simulink library "Transmission_Lib"  (R2025a)
settings: Solver=ode45  StartTime=0.0  StopTime=10.0  RelTol=1e-3  EnableMultiTasking=on
undefined symbols (not defined in the file): DCT_Param
libraries: fl_lib x45, nesl_utility x25, sdl_lib x18
(part 2 of 2)

== system Transmission_Lib/Detailed/Gears/Actu 6 ==
  p : Inport
  Actuation force (N) : Gain  Gain=10  SaturateOnIntegerOverflow=on  OutDataTypeStr=Inherit: Same as input  ParamDataTypeStr=Inherit: Same as input
  Ideal Force Source : fl_lib/Mechanical/Mechanical Sources/Ideal Force Source
  Mass : fl_lib/Mechanical/Translational Elements/Mass  mass=0.5 kg  num_ports=foundation.enum.numPorts2.one  v_specify=on  v_priority=High  v=0 m/s  v_nominal_specify=off  v_nominal_value=1  v_nominal_unit=m/s  f_specify=off  f_priority=High  f=0 N  f_nominal_specify=off  f_nominal_value=1  f_nominal_unit=N
  Mechanical Translational Reference : fl_lib/Mechanical/Translational Elements/Mechanical Translational Reference
  Rate Transition : RateTransition
  Simulink-PS Converter : nesl_utility/Simulink-PS Converter  PhysicalDomain=network_engine_domain  SubClassName=ps_input  LeftPortType=input  RightPortType=output  PseudoPeriodic=off  Frequencies=[]  NoiseDistribution=none  NoiseParameters=[]  Unit=1  AffineConversion=off  FilteringAndDerivatives=zero  SimscapeFilterOrder=1  InputFilterTimeConstant=0.005  UdotUserProvided=0
  S : PMIOPort  Side=Right
  wires:
  Rate Transition/1 -> Simulink-PS Converter/1
  Actuation force (N)/1 -> Rate Transition/1
  p/1 -> Actuation force (N)/1
  connections:
  Simulink-PS Converter/RConn1 -- Ideal Force Source/RConn1
  Mass/LConn1 -- S/RConn1 -- Ideal Force Source/LConn1
  Ideal Force Source/RConn2 -- Mechanical Translational Reference/LConn1

== system Transmission_Lib/Detailed/Gears/Actu R ==
  p : Inport
  Actuation force (N) : Gain  Gain=10  SaturateOnIntegerOverflow=on  OutDataTypeStr=Inherit: Same as input  ParamDataTypeStr=Inherit: Same as input
  Ideal Force Source : fl_lib/Mechanical/Mechanical Sources/Ideal Force Source
  Mass : fl_lib/Mechanical/Translational Elements/Mass  mass=0.5 kg  num_ports=foundation.enum.numPorts2.one  v_specify=on  v_priority=High  v=0 m/s  v_nominal_specify=off  v_nominal_value=1  v_nominal_unit=m/s  f_specify=off  f_priority=High  f=0 N  f_nominal_specify=off  f_nominal_value=1  f_nominal_unit=N
  Mechanical Translational Reference : fl_lib/Mechanical/Translational Elements/Mechanical Translational Reference
  Rate Transition : RateTransition
  Simulink-PS Converter : nesl_utility/Simulink-PS Converter  PhysicalDomain=network_engine_domain  SubClassName=ps_input  LeftPortType=input  RightPortType=output  PseudoPeriodic=off  Frequencies=[]  NoiseDistribution=none  NoiseParameters=[]  Unit=1  AffineConversion=off  FilteringAndDerivatives=zero  SimscapeFilterOrder=1  InputFilterTimeConstant=0.005  UdotUserProvided=0
  S : PMIOPort  Side=Right
  wires:
  p/1 -> Actuation force (N)/1
  Actuation force (N)/1 -> Rate Transition/1
  Rate Transition/1 -> Simulink-PS Converter/1
  connections:
  Ideal Force Source/RConn2 -- Mechanical Translational Reference/LConn1
  Ideal Force Source/LConn1 -- S/RConn1 -- Mass/LConn1
  Simulink-PS Converter/RConn1 -- Ideal Force Source/RConn1

== system Transmission_Lib/Detailed/Gears/Losses Off ==

== system Transmission_Lib/Detailed/Gears/Losses On ==

== system Transmission_Lib/Detailed/Gears/Sensing1 ==
  Ideal Rotational Motion Sensor : fl_lib/Mechanical/Mechanical Sensors/Ideal Rotational Motion Sensor  reference=foundation.enum.MeasurementReference.difference  acceleration_port=false  velocity_port=true  position_port=true  wrap_angle=simscape.enum.onoff.off  offset=0 rad
  Integrator : Integrator
  Mechanical Rotational Reference : fl_lib/Mechanical/Rotational Elements/Mechanical Rotational Reference
  PS-Simulink Converter : nesl_utility/PS-Simulink Converter  PhysicalDomain=network_engine_domain  SubClassName=ps_output  LeftPortType=input  RightPortType=output  PseudoPeriodic=off  Frequencies=[]  VectorFormat=1-D array  Unit=1  AffineConversion=off
  S : PMIOPort  Side=Left
  tag scope: DCT_Inp_Sh_Odd_Ang=global
  wires:
  Integrator/1 -> [DCT_Inp_Sh_Odd_Ang]
  PS-Simulink Converter/1 -> Integrator/1
  connections:
  Mechanical Rotational Reference/LConn1 -- Ideal Rotational Motion Sensor/RConn1
  PS-Simulink Converter/LConn1 -- Ideal Rotational Motion Sensor/RConn3
  S/RConn1 -- Ideal Rotational Motion Sensor/LConn1

== system Transmission_Lib/Detailed/Gears/Sensing10 ==
  PS-Simulink Converter : nesl_utility/PS-Simulink Converter  PhysicalDomain=network_engine_domain  SubClassName=ps_output  LeftPortType=input  RightPortType=output  PseudoPeriodic=off  Frequencies=[]  VectorFormat=1-D array  Unit=1  AffineConversion=off
  S : PMIOPort  Side=Left
  tag scope: DCT_ClR_Disp=global
  wires:
  PS-Simulink Converter/1 -> [DCT_ClR_Disp]
  connections:
  S/RConn1 -- PS-Simulink Converter/LConn1

== system Transmission_Lib/Detailed/Gears/Sensing2 ==
  Ideal Rotational Motion Sensor : fl_lib/Mechanical/Mechanical Sensors/Ideal Rotational Motion Sensor  reference=foundation.enum.MeasurementReference.difference  acceleration_port=false  velocity_port=true  position_port=true  wrap_angle=simscape.enum.onoff.off  offset=0 rad
  Integrator : Integrator
  Mechanical Rotational Reference : fl_lib/Mechanical/Rotational Elements/Mechanical Rotational Reference
  PS-Simulink Converter : nesl_utility/PS-Simulink Converter  PhysicalDomain=network_engine_domain  SubClassName=ps_output  LeftPortType=input  RightPortType=output  PseudoPeriodic=off  Frequencies=[]  VectorFormat=1-D array  Unit=1  AffineConversion=off
  S : PMIOPort  Side=Left
  tag scope: DCT_Inp_Sh_Even_Ang=global
  wires:
  Integrator/1 -> [DCT_Inp_Sh_Even_Ang]
  PS-Simulink Converter/1 -> Integrator/1
  connections:
  S/RConn1 -- Ideal Rotational Motion Sensor/LConn1
  PS-Simulink Converter/LConn1 -- Ideal Rotational Motion Sensor/RConn3
  Mechanical Rotational Reference/LConn1 -- Ideal Rotational Motion Sensor/RConn1

== system Transmission_Lib/Detailed/Gears/Sensing3 ==
  Ideal Rotational Motion Sensor : fl_lib/Mechanical/Mechanical Sensors/Ideal Rotational Motion Sensor  reference=foundation.enum.MeasurementReference.difference  acceleration_port=false  velocity_port=true  position_port=true  wrap_angle=simscape.enum.onoff.off  offset=0 rad
  Integrator : Integrator
  Mechanical Rotational Reference : fl_lib/Mechanical/Rotational Elements/Mechanical Rotational Reference
  PS-Simulink Converter : nesl_utility/PS-Simulink Converter  PhysicalDomain=network_engine_domain  SubClassName=ps_output  LeftPortType=input  RightPortType=output  PseudoPeriodic=off  Frequencies=[]  VectorFormat=1-D array  Unit=1  AffineConversion=off
  S : PMIOPort  Side=Left
  tag scope: DCT_Out_Sh_Even_Ang=global
  wires:
  Integrator/1 -> [DCT_Out_Sh_Even_Ang]
  PS-Simulink Converter/1 -> Integrator/1
  connections:
  S/RConn1 -- Ideal Rotational Motion Sensor/LConn1
  PS-Simulink Converter/LConn1 -- Ideal Rotational Motion Sensor/RConn3
  Mechanical Rotational Reference/LConn1 -- Ideal Rotational Motion Sensor/RConn1

== system Transmission_Lib/Detailed/Gears/Sensing4 ==
  PS-Simulink Converter : nesl_utility/PS-Simulink Converter  PhysicalDomain=network_engine_domain  SubClassName=ps_output  LeftPortType=input  RightPortType=output  PseudoPeriodic=off  Frequencies=[]  VectorFormat=1-D array  Unit=1  AffineConversion=off
  S : PMIOPort  Side=Left
  tag scope: DCT_Cl1_Disp=global
  wires:
  PS-Simulink Converter/1 -> [DCT_Cl1_Disp]
  connections:
  S/RConn1 -- PS-Simulink Converter/LConn1

== system Transmission_Lib/Detailed/Gears/Sensing5 ==
  PS-Simulink Converter : nesl_utility/PS-Simulink Converter  PhysicalDomain=network_engine_domain  SubClassName=ps_output  LeftPortType=input  RightPortType=output  PseudoPeriodic=off  Frequencies=[]  VectorFormat=1-D array  Unit=1  AffineConversion=off
  S : PMIOPort  Side=Left
  tag scope: DCT_Cl2_Disp=global
  wires:
  PS-Simulink Converter/1 -> [DCT_Cl2_Disp]
  connections:
  S/RConn1 -- PS-Simulink Converter/LConn1

== system Transmission_Lib/Detailed/Gears/Sensing6 ==
  PS-Simulink Converter : nesl_utility/PS-Simulink Converter  PhysicalDomain=network_engine_domain  SubClassName=ps_output  LeftPortType=input  RightPortType=output  PseudoPeriodic=off  Frequencies=[]  VectorFormat=1-D array  Unit=1  AffineConversion=off
  S : PMIOPort  Side=Left
  tag scope: DCT_Cl3_Disp=global
  wires:
  PS-Simulink Converter/1 -> [DCT_Cl3_Disp]
  connections:
  S/RConn1 -- PS-Simulink Converter/LConn1

== system Transmission_Lib/Detailed/Gears/Sensing7 ==
  PS-Simulink Converter : nesl_utility/PS-Simulink Converter  PhysicalDomain=network_engine_domain  SubClassName=ps_output  LeftPortType=input  RightPortType=output  PseudoPeriodic=off  Frequencies=[]  VectorFormat=1-D array  Unit=1  AffineConversion=off
  S : PMIOPort  Side=Left
  tag scope: DCT_Cl4_Disp=global
  wires:
  PS-Simulink Converter/1 -> [DCT_Cl4_Disp]
  connections:
  S/RConn1 -- PS-Simulink Converter/LConn1

== system Transmission_Lib/Detailed/Gears/Sensing8 ==
  PS-Simulink Converter : nesl_utility/PS-Simulink Converter  PhysicalDomain=network_engine_domain  SubClassName=ps_output  LeftPortType=input  RightPortType=output  PseudoPeriodic=off  Frequencies=[]  VectorFormat=1-D array  Unit=1  AffineConversion=off
  S : PMIOPort  Side=Left
  tag scope: DCT_Cl5_Disp=global
  wires:
  PS-Simulink Converter/1 -> [DCT_Cl5_Disp]
  connections:
  S/RConn1 -- PS-Simulink Converter/LConn1

== system Transmission_Lib/Detailed/Gears/Sensing9 ==
  PS-Simulink Converter : nesl_utility/PS-Simulink Converter  PhysicalDomain=network_engine_domain  SubClassName=ps_output  LeftPortType=input  RightPortType=output  PseudoPeriodic=off  Frequencies=[]  VectorFormat=1-D array  Unit=1  AffineConversion=off
  S : PMIOPort  Side=Left
  tag scope: DCT_Cl6_Disp=global
  wires:
  PS-Simulink Converter/1 -> [DCT_Cl6_Disp]
  connections:
  S/RConn1 -- PS-Simulink Converter/LConn1

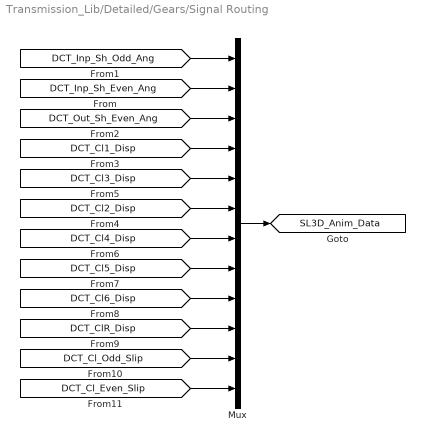
== system Transmission_Lib/Detailed/Gears/Signal Routing ==
  Mux : Mux  Inputs=12
  tag scope: SL3D_Anim_Data=global
  wires:
  [DCT_Cl_Even_Slip] -> Mux/12
  [DCT_Cl_Odd_Slip] -> Mux/11
  [DCT_ClR_Disp] -> Mux/10
  [DCT_Cl6_Disp] -> Mux/9
  [DCT_Cl5_Disp] -> Mux/8
  [DCT_Cl4_Disp] -> Mux/7
  [DCT_Cl2_Disp] -> Mux/6
  [DCT_Cl3_Disp] -> Mux/5
  [DCT_Cl1_Disp] -> Mux/4
  [DCT_Out_Sh_Even_Ang] -> Mux/3
  [DCT_Inp_Sh_Odd_Ang] -> Mux/1
  [DCT_Inp_Sh_Even_Ang] -> Mux/2
  Mux/1 -> [SL3D_Anim_Data]

== system Transmission_Lib/Abstracted/Gears/Ratio Selection/Lag Filter with IC ==
  In : Inport
  Gain : Gain  Gain=1/b
  Integrator : Integrator  InitialCondition=x_initial*b
  Sum : Sum  Inputs=|+-  InputSameDT=on  SaturateOnIntegerOverflow=on  OutDataTypeStr=Inherit: Same as first input
  Out : Outport  VectorParamsAs1DForOutWhenUnconnected=off
  wires:
  Gain/1 -> Out/1, Sum/2
  Integrator/1 -> Gain/1
  In/1 -> Sum/1
  Sum/1 -> Integrator/1

== system Transmission_Lib/Detailed/Clutches/Slip sensor 1/Sensing4 ==
  S : Inport
  tag scope: DCT_Cl_Odd_Slip=global
  wires:
  S/1 -> [DCT_Cl_Odd_Slip]

== system Transmission_Lib/Detailed/Clutches/Slip sensor 2/Sensing4 ==
  S : Inport
  tag scope: DCT_Cl_Even_Slip=global
  wires:
  S/1 -> [DCT_Cl_Even_Slip]
